simulink model "PEM_Plant"  (R2023b)
settings: Solver=ode23t  StartTime=0.0  StopTime=1  RelTol=1e-3
PreLoadFcn:
  | if ~exist('SIM_A','var'), SIM_A = 100; end;
  | if ~exist('SIM_N','var'), SIM_N =  20; end;
  | if ~exist('SIM_J','var'), SIM_J =   1; end;
  | if ~exist('SIM_T','var'), SIM_T =  70; end;
  | if ~exist('SIM_P','var'), SIM_P =  10; end
undefined symbols (not defined in the file or in its folder): SIM_A, SIM_J, SIM_N, SIM_P, SIM_T
settings Model: Creator=Admin  LastModifiedBy=Admin

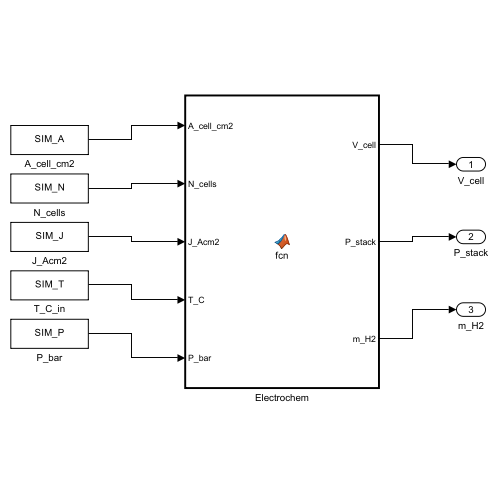
[thumbnail: Simulink's stored preview of the top-level diagram]
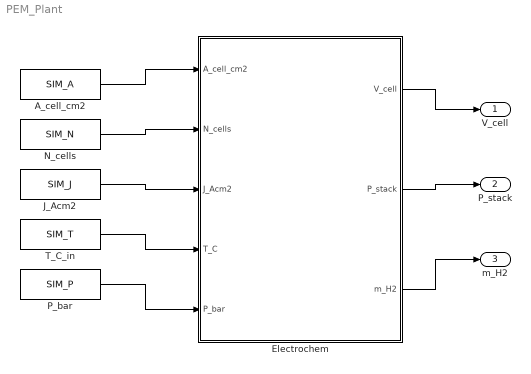
== system PEM_Plant ==
  A_cell_cm2 : Constant  Value=SIM_A
  Electrochem : MATLAB Function  TreatAsAtomicUnit=on
  J_Acm2 : Constant  Value=SIM_J
  N_cells : Constant  Value=SIM_N
  P_bar : Constant  Value=SIM_P
  T_C_in : Constant  Value=SIM_T
  V_cell : Outport
  P_stack : Outport  Port=2
  m_H2 : Outport  Port=3
  wires:
  A_cell_cm2/1 -> Electrochem/1(A_cell_cm2)
  N_cells/1 -> Electrochem/2(N_cells)
  J_Acm2/1 -> Electrochem/3(J_Acm2)
  T_C_in/1 -> Electrochem/4(T_C)
  P_bar/1 -> Electrochem/5(P_bar)
  Electrochem/1(V_cell) -> V_cell/1
  Electrochem/2(P_stack) -> P_stack/1
  Electrochem/3(m_H2) -> m_H2/1

== matlab function PEM_Plant/Electrochem ==
  data: A_cell_cm2 input; V_cell output; N_cells input; J_Acm2 input; T_C input; P_bar input; P_stack output; m_H2 output
function [V_cell, P_stack, m_H2] = fcn(A_cell_cm2, N_cells, J_Acm2, T_C, P_bar)
    F      = 96485;
    R      = 8.314;
    M_H2   = 2.016e-3;
    E_rev  = 1.42;
    alpha  = 0.448938;
    j0     = 5.428292e-02;
    R_ohm  = 0.169475;
    k_conc = 4e-6;
    n_e    = 2;
    T_K    = T_C + 273.15;
    E_rev_T = E_rev - 0.0009*(T_C - 75);
    f = R*T_K/(alpha*n_e*F);
    eta_act  = f * asinh(J_Acm2/(2*j0));
    eta_ohm  = R_ohm * J_Acm2;
    eta_conc = k_conc * J_Acm2^2;
    V_nernst = (R*T_K/(2*F)) * log(P_bar/1.0);
    V_cell   = E_rev_T + eta_act + eta_ohm + eta_conc + V_nernst;
    I_stack  = J_Acm2 * A_cell_cm2;
    P_stack  = N_cells * V_cell * I_stack;
    m_H2     = N_cells * I_stack / (2*F) * M_H2;
end
